simulink model "implcmd_can_unpack"  (R2026b)
settings: Solver=VariableStepAuto
undefined symbols (not defined in the file or in its folder): Ts
libraries: simulink x3, svdutilitieslib x1
settings Model: Creator=aomar  LastModifiedBy=aomar

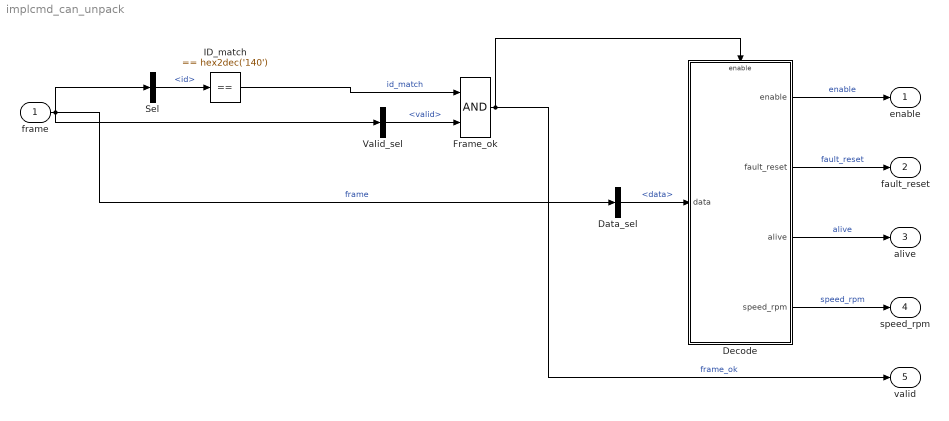
== system implcmd_can_unpack ==
  frame : Inport  OutDataTypeStr=Bus: Bus_CanFrame8  SampleTime=Ts.can_slow
  Data_sel : BusSelector  OutputSignals=data
  Decode : Subsystem  TreatAsAtomicUnit=on
  Frame_ok : Logic  AllPortsSameDT=off  OutDataTypeStr=boolean
  ID_match : simulink/Logic and Bit Operations/Compare To Constant  relop===  const=hex2dec('140')  OutDataTypeStr=boolean
  Sel : BusSelector  OutputSignals=id
  Valid_sel : BusSelector  OutputSignals=valid
  enable : Outport
  fault_reset : Outport  Port=2
  alive : Outport  Port=3
  speed_rpm : Outport  Port=4
  valid : Outport  Port=5  OutDataTypeStr=boolean
  wires:
  frame/1 -> Data_sel/1, Sel/1, Valid_sel/1  "frame"
  Sel/1 -> ID_match/1  "<id>"
  ID_match/1 -> Frame_ok/1  "id_match"
  Valid_sel/1 -> Frame_ok/2  "<valid>"
  Frame_ok/1 -> valid/1, Decode/Enable  "frame_ok"
  Data_sel/1 -> Decode/1(data)  "<data>"
  Decode/1(enable) -> enable/1  "enable"
  Decode/2(fault_reset) -> fault_reset/1  "fault_reset"
  Decode/3(alive) -> alive/1  "alive"
  Decode/4(speed_rpm) -> speed_rpm/1  "speed_rpm"

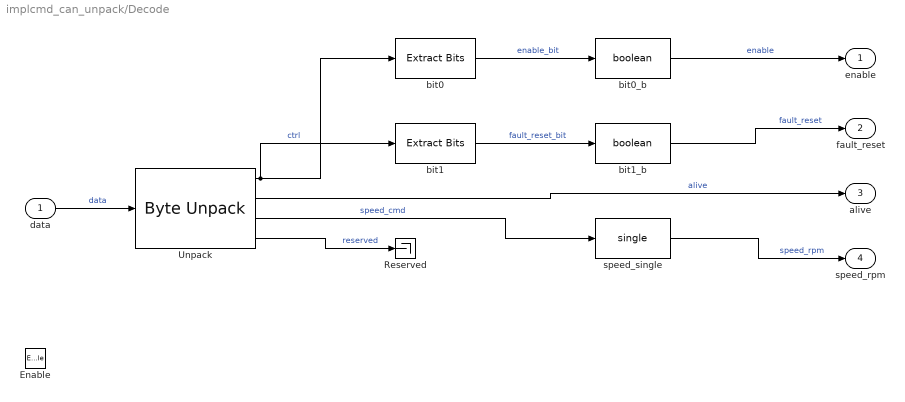
== system implcmd_can_unpack/Decode ==
  data : Inport
  Enable : EnablePort
  Reserved : Terminator
  Unpack : svdutilitieslib/Byte Unpack  dimensions={1,1,1,4}  datatypes={'uint8','uint8','int16','uint8'}  byteAlign=1  blockPlatform=arduinoert
      settings: LibrarySourceBlock=mcblib/Signal Management/Byte Unpack
  bit0 : simulink/Logic and Bit Operations/Extract Bits  bitsToExtract=Range of bits  numBits=8  bitIdxRange=[0 0]  outScalingMode=Treat bit field as an integer
  bit0_b : DataTypeConversion  OutDataTypeStr=boolean  RndMeth=Nearest
  bit1 : simulink/Logic and Bit Operations/Extract Bits  bitsToExtract=Range of bits  numBits=8  bitIdxRange=[1 1]  outScalingMode=Treat bit field as an integer
  bit1_b : DataTypeConversion  OutDataTypeStr=boolean  RndMeth=Nearest
  speed_single : DataTypeConversion  OutDataTypeStr=single  RndMeth=Nearest
  enable : Outport  OutDataTypeStr=boolean  InitialOutput=0
  fault_reset : Outport  Port=2  OutDataTypeStr=boolean  InitialOutput=0
  alive : Outport  Port=3  OutDataTypeStr=uint8  InitialOutput=0
  speed_rpm : Outport  Port=4  OutDataTypeStr=single  InitialOutput=0
  wires:
  data/1 -> Unpack/1  "data"
  Unpack/1 -> bit0/1, bit1/1  "ctrl"
  Unpack/2 -> alive/1  "alive"
  Unpack/3 -> speed_single/1  "speed_cmd"
  Unpack/4 -> Reserved/1  "reserved"
  bit0/1 -> bit0_b/1  "enable_bit"
  bit1/1 -> bit1_b/1  "fault_reset_bit"
  bit0_b/1 -> enable/1  "enable"
  bit1_b/1 -> fault_reset/1  "fault_reset"
  speed_single/1 -> speed_rpm/1  "speed_rpm"
